simulink model "Open_loop_VSI_fed_3_phase_induction_motor_drive_SPWM"  (R2024a)
settings: Solver=VariableStepAuto  StartTime=0.0  StopTime=5  RelTol=1e-3
libraries: spsIGBTLib x6, spsAsynchronousMachineSIUnitsLib x1, spsDCVoltageSourceLib x1, sps_lib x1
settings Model: Creator=haris  LastModifiedBy=haris

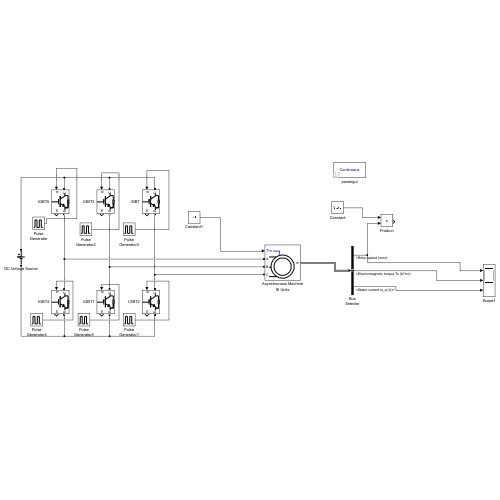
[thumbnail: Simulink's stored preview of the top-level diagram]
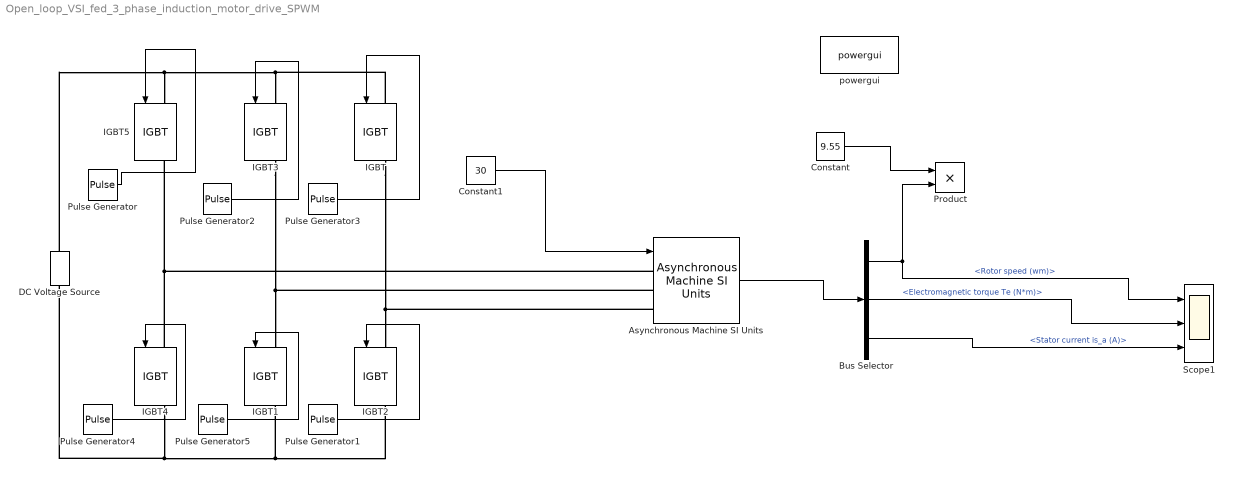
== system Open_loop_VSI_fed_3_phase_induction_motor_drive_SPWM ==
  Asynchronous Machine SI Units : spsAsynchronousMachineSIUnitsLib/Asynchronous Machine SI Units  RotorType=Squirrel-cage  PresetModel=No  MechanicalLoad=Torque Tm  ShowDetailedParameters=on  ReferenceFrame=Rotor  Units=SI  MeasurementBus=off  NominalParameters=[1.845e+04 400 50]  VoltageRatio=1  Stator=[0.5968 0.0003495]  Rotor=[0.6258 0.005473]  Cage1=[0.4155 0.002066]  Cage2=[0.4168 0.0003495]  Lm=0.0354  Mechanical=[0.05 0.005879 2]  PolePairs=2  InitialConditions=[0 0 0 0 0 0 0 0]  SimulateSaturation=off  Saturation=[14.03593122, 27.81365428, 53.79336849, 72.68890987, 97.98006896, 148.6815601, 215.7428561, 302.9841135, 428.7778367 ; 230, 322, 414, 460, 506, 552, 598, 644, 690]  LoadFlowParameters=1492000  TsPowergui=0  TsBlock=-1  IterativeModel=Trapezoidal non iterative  IterativeDiscreteModel=Trapezoidal non iterative  Pmec=1.492e+006
  Bus Selector : BusSelector  OutputSignals=Mechanical.Rotor speed (wm),Mechanical.Electromagnetic torque Te (N*m),Stator measurements.Stator current is_a (A)
  Constant : Constant  Value=9.55
  Constant1 : Constant  Value=30
  DC Voltage Source : spsDCVoltageSourceLib/DC Voltage Source  Amplitude=400  Measurements=None
  IGBT{,1..5} (6 alike) : spsIGBTLib/IGBT  Ron=0.001  Lon=0  Vf=1  Tf=1e-6  Tt=2e-6  IC=0  Rs=1e5  Cs=inf  Measurements=on
  Product : Product
  Pulse Generator : DiscretePulseGenerator  PulseType=Time based  Period=0.02  PulseWidth=33
  Pulse Generator1 : DiscretePulseGenerator  PulseType=Time based  Period=0.02  PulseWidth=33  PhaseDelay=0.0033
  Pulse Generator2 : DiscretePulseGenerator  PulseType=Time based  Period=0.02  PulseWidth=33  PhaseDelay=0.0066
  Pulse Generator3 : DiscretePulseGenerator  PulseType=Time based  Period=0.02  PulseWidth=33  PhaseDelay=0.0133
  Pulse Generator4 : DiscretePulseGenerator  PulseType=Time based  Period=0.02  PulseWidth=33  PhaseDelay=0.01
  Pulse Generator5 : DiscretePulseGenerator  PulseType=Time based  Period=0.02  PulseWidth=33  PhaseDelay=0.0166
  Scope1 : Scope  NumInputPorts=3
  powergui : sps_lib/powergui  Priority=1  SimulationMode=Continuous  SampleTime=50e-6  frequency=60  Iterations=50  frequencyindice=50  Pbase=100e6  ErrMax=1e-4  UnitsV=kV  UnitsW=MW  buscounter=0  FunctionMessages=off  echomessages=off  EnableUseOfTLC=off  CurrentSourceSwitches=off  DisableSnubberDevices=off  DisableRonSwitches=off  DisableVfSwitches=off  DisplayEquations=off  AutomaticDiscreteSolvers=off  SolverType=Tustin/Backward Euler (TBE)  Interpol=off  ExternalGateDelay=off  methode=off  Ts=100  x0status=blocks  SPID=on  SwTol=0  HookPort=off  NonlinearTolerance=1e-4  nMaxIteration=100  ContinueOnMaxIteration=off  RestoreLinks=warning  ResistiveCurrentMeasurement=off  Frange=[0:2:500]  Ylog=off  Xlog=on  ShowGrid=off  save=off  variable=ZData  structure=0  ZoomFFT=off  StartTime=0.0  cycles=1  DisplayStyle=1  fundamental=60  FreqAxis=off  MaxFrequency=1000  frequencyindicesteady=1  RmsSteady=1  display=off
  wires:
  Pulse Generator/1 -> IGBT5/1
  Pulse Generator2/1 -> IGBT3/1
  Pulse Generator3/1 -> IGBT/1
  Pulse Generator4/1 -> IGBT4/1
  Pulse Generator5/1 -> IGBT1/1
  Pulse Generator1/1 -> IGBT2/1
  Constant1/1 -> Asynchronous Machine SI Units/1
  Asynchronous Machine SI Units/1 -> Bus Selector/1
  Bus Selector/1 -> Scope1/1, Product/2  "<Rotor speed (wm)>"
  Constant/1 -> Product/1
  Bus Selector/2 -> Scope1/2  "<Electromagnetic torque Te (N*m)>"
  Bus Selector/3 -> Scope1/3  "<Stator current is_a (A)>"
  connections:
  IGBT4/LConn1 -- IGBT5/RConn1 -- Asynchronous Machine SI Units/LConn1
  IGBT3/RConn1 -- Asynchronous Machine SI Units/LConn2 -- IGBT1/LConn1
  IGBT/RConn1 -- Asynchronous Machine SI Units/LConn3 -- IGBT2/LConn1
  DC Voltage Source/RConn1 -- IGBT5/LConn1 -- IGBT/LConn1 -- IGBT3/LConn1
  IGBT4/RConn1 -- DC Voltage Source/LConn1 -- IGBT1/RConn1 -- IGBT2/RConn1
